simulink model "s20260910_config2torque_sim_chatgpt"  (R2025a)
settings: Solver=daessc  StartTime=0.0  StopTime=20  FixedStep=0.01  MaxStep=0.05  RelTol=1e-3  AbsTol=1e-3  EnableMultiTasking=on
undefined symbols (not defined in the file or in its folder): X, Y, Z
libraries: sm_lib x9, nesl_utility x4, snake_single_module_library_torque x1, slpidlib x1, simulink x1, spsSawtoothGeneratorLib x1, cstblocks x1
settings Model: Creator=dperera  LastModifiedBy=dperera
settings SolverCC: AutoScaleAbsTol=off  AlgebraicLoopSolver=TrustRegion  MaxZcPerStep=1.0
settings DataIOCC: LimitDataPoints=on  MaxDataPoints=10000
settings OptimizationCC: ReuseModelBlockBuffer=off  LifeSpan=inf
settings DebuggingCC: UnconnectedInputMsg=warning  UnconnectedOutputMsg=warning  UnconnectedLineMsg=warning  AllowSymbolicDim=off  SubsystemReferenceDiagnosticForUnitTest=warning  SFUnexpectedBacktrackingDiag=warning  SFNoUnconditionalDefaultTransitionDiag=warning  SFExecutionAtInitializationDiag=none  ArithmeticOperatorsInVariantConditions=warning
settings ModelReferenceCC: EnableRefExpFcnMdlSchedulingChecks=on
settings SFSimCC: SimUseLocalCustomCode=off  CustomCodeUndefinedFunction=UseInterfaceOnly
settings RTWCC: RTWUseLocalCustomCode=off  GPUComputeCapability=3.5  DLArmComputeVersion=19.05
settings CodeAppCC: StateflowObjectComments=on
settings GRTTargetCC: TargetLangStandard=C89/C90 (ANSI)
settings ConfigComp: CovMetricSettings=dw  CovSaveCumulativeToWorkspaceVar=on  CovSaveSingleToWorkspaceVar=on  CovExternalEMLEnable=off  CovSFcnEnable=off
settings SimscapeCC: SimscapeLogType=all  SimscapeLogSimulationStatistics=on  SimscapeLogDataHistory=10000.0

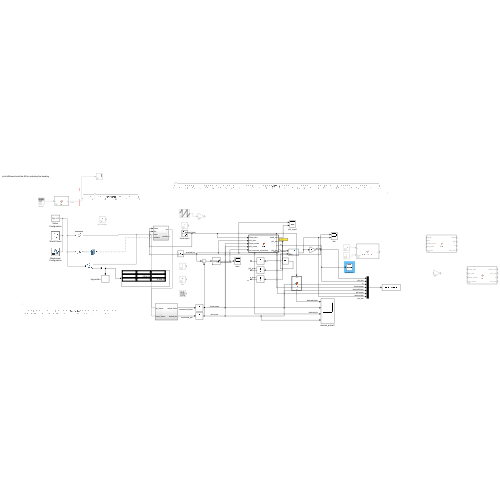
[thumbnail: Simulink's stored preview of the top-level diagram]
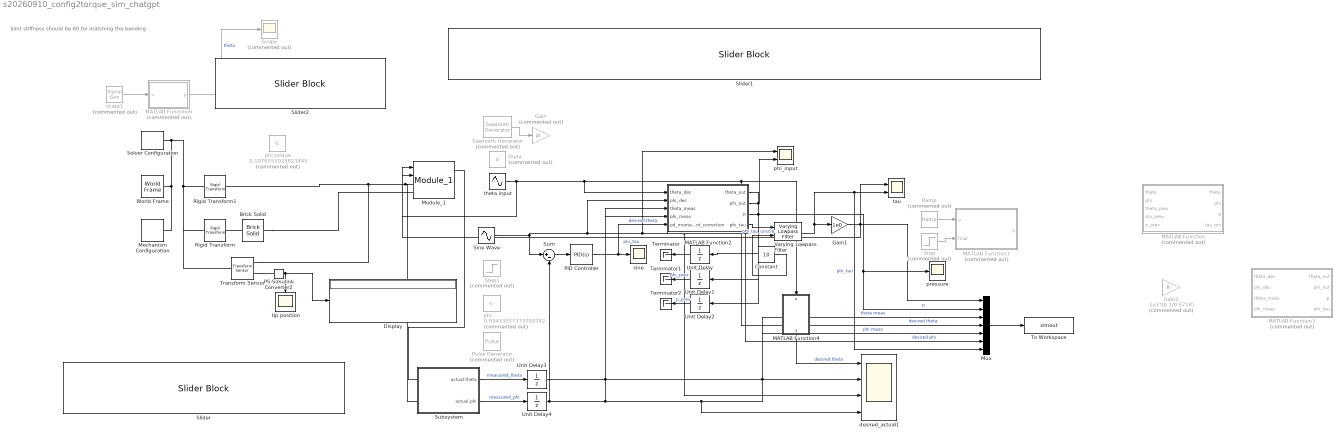
== system s20260910_config2torque_sim_chatgpt ==
  note: joint stiffness should be 60 for matching the bending
  Brick Solid : sm_lib/Body Elements/Brick Solid  BrickDimensions=[0.5 0.5 0.01]  BrickDimensionsUnits=m  ExportEntireGeometry=on  InertiaType=CalculateFromGeometry  BasedOnType=Density  Density=1000  DensityUnits=kg/m^3  Mass=1  MassUnits=kg  CenterOfMass=[0 0 0]  CenterOfMassUnits=m  MomentsOfInertia=[1 1 1]  MomentsOfInertiaUnits=kg*m^2  ProductsOfInertia=[0 0 0]  ProductsOfInertiaUnits=kg*m^2  GraphicType=FromGeometry  MarkerShape=Sphere  MarkerSize=10  GraphicVisPropType=SimpleVisualProperties  GraphicDiffuseColor=[0.5 0.5 0.5]  GraphicOpacity=1  GraphicSpecularColor=[0.5 0.5 0.5 1.0]  GraphicAmbientColor=[0.15 0.15 0.15 1.0]  GraphicEmissiveColor=[0.0 0.0 0.0 1.0]  GraphicShininess=75  DoExposeReferenceFrame=on  SerializedFrames=<Frames/>
  Constant : Constant  Value=10
  Display : Display
  Gain : Gain  Commented=on  Gain=pi
  Gain1 : Gain  Gain=1e0
  Gain2 : Gain  Commented=on  Gain=1e1*(0.1/0.5714)
  MATLAB Function : MATLAB Function  Commented=on  TreatAsAtomicUnit=on
  MATLAB Function1 : MATLAB Function  Commented=on  TreatAsAtomicUnit=on
  MATLAB Function2 : MATLAB Function  TreatAsAtomicUnit=on
  MATLAB Function3 : MATLAB Function  Commented=on  TreatAsAtomicUnit=on
  MATLAB Function4 : MATLAB Function  TreatAsAtomicUnit=on
  MATLAB Function6 : MATLAB Function  Commented=on  TreatAsAtomicUnit=on
  Mechanism Configuration : sm_lib/Utilities/Mechanism Configuration  UniformGravity=Constant  GravityVector=[0 0 -9.80665]  GravityVectorUnits=m/s^2  LinearizationDelta=0.001  JointModeTransitionNonlinearIterations=2
  Module_1 : snake_single_module_library_torque/Module_1  SystemSampleTime=-1  VariantActivationTime=update diagram  EmptyChoice=off  PassThrough=off  PassThroughVariantControl=(default)  EmptyChoiceVariantControl=(default)  AllowFlexibleInterface=on  Latency=0  AutoFrameSizeCalculation=off
  Mux : Mux  Inputs=7
  PID Controller : slpidlib/PID Controller  Controller=PID  Form=Parallel  TimeDomain=Continuous-time  UseExternalTs=off  SampleTime=-1  IntegratorMethod=Forward Euler  FilterMethod=Forward Euler  ControllerParametersSource=internal  P=0.3  I=0.1  UseKiTs=off  D=0.0001  UseExternalDerivativeSource=off  N=100  UseFilter=on  TunerSelectOption=Frequency Response Based  InitialConditionSource=internal  InitialConditionForIntegrator=0  InitialConditionForFilter=0  DifferentiatorICPrevScaledInput=0  ExternalReset=none  TrackingMode=off  Kt=1  LimitOutput=on  SatLimitsSource=internal  UpperSaturationLimit=inf  LowerSaturationLimit=-inf  LinearizeAsGain=on  AntiWindupMode=back-calculation  Kb=1  LimitIntegrator=off  UpperIntegratorSaturationLimit=inf  LowerIntegratorSaturationLimit=-inf  POutMin=[]  POutMax=[]  IOutMin=[]  IOutMax=[]  DOutMin=[]  DOutMax=[]  NOutMin=[]  NOutMax=[]  SumOutMin=[]  SumOutMax=[]  SaturationOutMin=[]  SaturationOutMax=[]  PParamMin=[]  PParamMax=[]  IParamMin=[]  IParamMax=[]  DParamMin=[]  DParamMax=[]  NParamMin=[]  NParamMax=[]  KbParamMin=[]  KbParamMax=[]  KtParamMin=[]  KtParamMax=[]  KbOutMin=[]  KbOutMax=[]  KtOutMin=[]  KtOutMax=[]  IntegratorOutMin=[]  IntegratorOutMax=[]  FilterOutMin=[]  FilterOutMax=[]  SumI1OutMin=[]  SumI1OutMax=[]  SumI2OutMin=[]  SumI2OutMax=[]  SumI3OutMin=[]  SumI3OutMax=[]  SumI4OutMin=[]  SumI4OutMax=[]  SumDOutMin=[]  SumDOutMax=[]  DifferentiatorOutMin=[]  DifferentiatorOutMax=[]  FilterDiffOutCoefMin=[]  FilterDiffOutCoefMax=[]  ReciprocalOutMin=[]  ReciprocalOutMax=[]  SumDenOutMin=[]  SumDenOutMax=[]  SumNumOutMin=[]  SumNumOutMax=[]  DivideOutMin=[]  DivideOutMax=[]  UdiffTsProdOutMin=[]  UdiffTsProdOutMax=[]  NTsProdOutMin=[]  NTsProdOutMax=[]  UintegralTsProdOutMin=[]  UintegralTsProdOutMax=[]  UngainTsProdOutMin=[]  UngainTsProdOutMax=[]  ClampingZeroOutDataTypeStr=Inherit: Inherit via back propagation  ClampingZeroOutMin=[]  ClampingZeroOutMax=[]  FilterDenConstantOutDataTypeStr=Inherit: Inherit via back propagation  FilterDenConstantOutMin=[]  FilterDenConstantOutMax=[]  PCopyOutDataTypeStr=Inherit: Inherit via back propagation  PCopyOutMin=[]  PCopyOutMax=[]  NCopyOutDataTypeStr=Inherit: Inherit via back propagation  NCopyOutMin=[]  NCopyOutMax=[]  IntegratorContinuousStateAttributes=''  IntegratorStateMustResolveToSignalObject=off  IntegratorRTWStateStorageClass=Auto  FilterContinuousStateAttributes=''  FilterStateMustResolveToSignalObject=off  FilterRTWStateStorageClass=Auto  ParallelPVariant=InternalParameters  IdealPVariant=Disabled  IVariant=InternalParameters  DVariant=InternalParameters  IntegratorVariant=Continuous  SatVariant=Enabled  AWVariant=BackCalculation  PCopyVariant=Disabled  TRVariant=Disabled  FdbkBlocksVariant=Forward  IdealPFdbkVariant=Disabled  SatFdbkVariant=Disabled  DerivativeFilterVariant=ContFilter  NVariant=InternalParameters  NCopyVariant=Disabled  FilterICVariant=InternalICsFilter  IntegratorICVariant=InternalICs  ExternalResetVariant=Disabled  TRSumVariant=Passthrough  SumFdbkVariant=Disabled  SumVariant=Sum_PID  TsampFilterVariant=InternalTs  TsampNgainVariant=Passthrough  TsampIntegralVariant=Disabled_SignalSpec  ExternalSaturationOutDataTypeStr=Inherit: Same as second input  DerivativeSourceVariant=ErrorSignal  PreIntVariant=InternalPreInt
  PS-Simulink Converter2 : nesl_utility/PS-Simulink Converter  PhysicalDomain=network_engine_domain  SubClassName=ps_output  LeftPortType=input  RightPortType=output  PseudoPeriodic=off  Frequencies=[]  VectorFormat=inherit  Unit=inherit  AffineConversion=off
  Pulse Generator : DiscretePulseGenerator  Commented=on  PulseType=Time based  Amplitude=pi/3  Period=4  PulseWidth=50  PhaseDelay=1
  Ramp : simulink/Sources/Ramp  Commented=on  slope=0.01*2*pi  start=1  InitialOutput=0.001
  Rigid Transform : sm_lib/Frames and Transforms/Rigid Transform  RotationMethod=None  FollAlignAxisA=+X  BaseAlignAxisA=+Y  FollAlignAxisB=+Y  BaseAlignAxisB=+Z  RotationStandardAxis=+Z  RotationAngle=0  RotationAngleUnits=deg  RotationArbitraryAxis=[0 0 1]  RotationSequenceAxes=FollowerAxes  RotationSequence=XYX  RotationSequenceAngles=[0 0 0]  RotationSequenceAnglesUnits=deg  RotationMatrix=[1 0 0;0 1 0;0 0 1]  Quaternion=[1 0 0 0]  TranslationMethod=StandardAxis  TranslationCartesianOffset=[0 0 0]  TranslationCartesianOffsetUnits=m  TranslationStandardAxis=+Z  TranslationStandardOffset=-0.03  TranslationStandardOffsetUnits=m  TranslationROffset=0  TranslationROffsetUnits=m  TranslationThetaOffset=0  TranslationThetaOffsetUnits=deg  TranslationZOffset=0  TranslationZOffsetUnits=m
  Rigid Transform1 : sm_lib/Frames and Transforms/Rigid Transform  RotationMethod=StandardAxis  FollAlignAxisA=+X  BaseAlignAxisA=+Y  FollAlignAxisB=+Y  BaseAlignAxisB=+Z  RotationStandardAxis=+X  RotationAngle=-pi/2  RotationAngleUnits=rad  RotationArbitraryAxis=[0 0 1]  RotationSequenceAxes=FollowerAxes  RotationSequence=XYX  RotationSequenceAngles=[0 0 0]  RotationSequenceAnglesUnits=deg  RotationMatrix=[1 0 0;0 1 0;0 0 1]  Quaternion=[1 0 0 0]  TranslationMethod=StandardAxis  TranslationCartesianOffset=[0 0 0]  TranslationCartesianOffsetUnits=m  TranslationStandardAxis=+Z  TranslationStandardOffset=0.5  TranslationStandardOffsetUnits=m  TranslationROffset=0  TranslationROffsetUnits=m  TranslationThetaOffset=0  TranslationThetaOffsetUnits=deg  TranslationZOffset=0  TranslationZOffsetUnits=m
  Sawtooth Generator : spsSawtoothGeneratorLib/Sawtooth Generator  Commented=on  Freq=0.5  Phase=180  Ts=0.001
  Scope : Scope  Commented=on
      settings: ActiveDisplayYMinimum=-3.3334127281449564  ActiveDisplayYMaximum=3.1584952199962761
  Sine Wave : Sin  Amplitude=pi/2-0.3  Bias=pi/2-0.3  Phase=3*pi/2  SampleTime=0
  Slider : SliderBlock  ScaleMin=-3.14  ScaleMax=6
  Slider1 : SliderBlock  ScaleMax=3.14
  Slider2 : SliderBlock  ScaleMax=0.5
  Solver Configuration : nesl_utility/Solver Configuration  PhysicalDomain=network_engine_domain  SubClassName=solver  LeftPortType=input  RightPortType=generic  Tones=[]  Harmonics=[]  SimulateNoise=off  Profile=off  UseLocalSampling=off  EnableSwitchedLinearOptims=on  FrequencyDomain=off  UseCCode=off  RelTol=0.001  AbsTol=1e-06  MinStep=1e-09  ToWorkspace=off  RevertToSquareIcSolve=off  NumHomotopyIterations=100  PhasorMode=off  PhasorModeNumHarmonics=1  ConsistencySolver=NEWTON_XTOL_AFTER_FTOL  IndexReductionMethod=DerivativeReplacement  DoDC=off  ResidualTolerance=1e-09  ConsistencyTolSource=GLOBAL  ConsistencyAbsTol=0.001  ConsistencyRelTol=0.001  ConsistencyTolFactor=0.001  UseLocalSolver=off  LocalSolverChoice=NE_BACKWARD_EULER_ADVANCER  ResolveIndetEquations=on  FunctionEvalNumThread=1  LocalSolverSampleTime=0.001  DoFixedCost=off  MaxNonlinIter=3  MaxModeIter=2  ComputeImpulses=off  ImpulseIterations=2  LinearAlgebra=Sparse  LinearAlgebraNumThread=0  EquationFormulation=NE_TIME_EF  DelaysMemoryBudget=1024  AutomaticFiltering=on  FilteringTimeConstant=0.001  PartitionStorageMethod=AS_NEEDED  PartitionMemoryBudget=1024  PartitionMethod=FAST  MultibodyUseLocalSolver=off  MultibodyLocalSolverChoice=ODE1  MultibodyLocalSolverSampleTime=0.001
  Step : Step  Commented=on  Time=2  SampleTime=0
  Step1 : Step  Commented=on  After=pi/3  SampleTime=0
  Subsystem : Subsystem
  Sum : Sum  Inputs=|+-
  Terminator : Terminator
  Terminator1 : Terminator
  Terminator2 : Terminator
  To Workspace : ToWorkspace  VariableName=simout  SaveFormat=Timeseries  SampleTime=-1
      settings: Save2DSignal=2-D array (concatenate along first dimension)
  Transform Sensor : sm_lib/Frames and Transforms/Transform Sensor  MeasurementFrame=World  RotationSequence=XYX  SenseAngle=off  SenseAxis=off  SenseQ=off  SenseR=on  SenseRotationSequence=off  SenseOmegaX=off  SenseOmegaY=off  SenseOmegaZ=off  SenseOmega=off  SenseQDot=off  SenseRDot=off  SenseRotationSequenceDot=off  SenseAlphaX=off  SenseAlphaY=off  SenseAlphaZ=off  SenseAlpha=off  SenseQDDot=off  SenseRDDot=off  SenseX=off  SenseY=off  SenseZ=off  SenseXYZ=off  SenseRad=off  SenseAzim=off  SenseDist=off  SenseInc=off  SenseXDot=off  SenseYDot=off  SenseZDot=off  SenseXYZDot=off  SenseRadDot=off  SenseAzimDot=off  SenseDistDot=off  SenseIncDot=off  SenseXDDot=off  SenseYDDot=off  SenseZDDot=off  SenseXYZDDot=off  SenseRadDDot=off  SenseAzimDDot=off  SenseDistDDot=off  SenseIncDDot=off
  Unit Delay : UnitDelay  InitialCondition=[0]  SampleTime=-1  HasFrameUpgradeWarning=on
  Unit Delay1 : UnitDelay  InitialCondition=0.0001  SampleTime=-1  HasFrameUpgradeWarning=on
  Unit Delay2 : UnitDelay  InitialCondition=[0.0001;0.01;0.001]  SampleTime=-1  HasFrameUpgradeWarning=on
  Unit Delay3 : UnitDelay  InitialCondition=[0]  SampleTime=-1  HasFrameUpgradeWarning=on
  Unit Delay4 : UnitDelay  InitialCondition=0.0001  SampleTime=-1  HasFrameUpgradeWarning=on
  Varying Lowpass Filter : cstblocks/Linear Parameter Varying/Varying Lowpass Filter  N=1
  World Frame : sm_lib/Frames and Transforms/World Frame
  desired_actual1 : Scope  NumInputPorts=4
      settings: ActiveDisplayYMinimum=-0.37614430678155741  ActiveDisplayYMaximum=3.3852987610340177  DataLoggingVariableName=ScopeData7
  phi : Constant  Commented=on  Value=0.03433257333758742
  phi torque : Constant  Commented=on  Value=0.1076555023923445
  phi_input : Scope  NumInputPorts=2
      settings: ActiveDisplayYMinimum=-0.36834079509334744  ActiveDisplayYMaximum=3.3160671558401278  DataLoggingVariableName=ScopeData3
  pressure : Scope
      settings: ActiveDisplayYMinimum=-30741.22465781157  ActiveDisplayYMaximum=510004.6447710325  DataLoggingVariableName=ScopeData4
  sine : Scope
      settings: ActiveDisplayYMinimum=-0.41740703510045596  ActiveDisplayYMaximum=3.0703490190244911  DataLoggingVariableName=ScopeData2
  tau : Scope  NumInputPorts=2
      settings: ActiveDisplayYMinimum=-0.07521570426510249  ActiveDisplayYMaximum=0.65254070404289077
  theta : Constant  Commented=on  Value=0
  theta input : Sin  Amplitude=pi-0.1  Frequency=0.1  SampleTime=0
  theta1 : SignalGenerator  Commented=on  WaveForm=sawtooth  Amplitude=pi  Frequency=0.1*2*pi  Units=rad/sec  VectorParams1D=off
  tip position : Scope
      settings: ActiveDisplayYMinimum=-1.2500000000000002  ActiveDisplayYMaximum=1.2500000000000004  DataLoggingVariableName=ScopeData5
  wires:
  Sawtooth Generator/1 -> Gain/1
  theta1/1 -> MATLAB Function6/1(u)
  MATLAB Function6/1(y) -> Scope/1  "theta"
  MATLAB Function2/1(theta_out) -> Unit Delay/1
  MATLAB Function2/2(phi_out) -> Unit Delay1/1, phi_input/2
  MATLAB Function2/3(p) -> Mux/2, pressure/1, Unit Delay2/1  "p"
  theta input/1 -> Mux/4, MATLAB Function4/1(u), MATLAB Function2/1(theta_des), Module_1/1  "desired theta"
  Ramp/1 -> MATLAB Function1/1(u)
  Step/1 -> MATLAB Function1/2(final)
  MATLAB Function4/1(y) -> desired_actual1/1  "desired theta"
  Gain1/1 -> Module_1/2, Mux/1, tau/1  "phi_tau"
  Sine Wave/1 -> desired_actual1/3, Mux/6, phi_input/1, MATLAB Function2/2(phi_des), Sum/1  "desired phi"
  Subsystem/1(actual theta) -> Unit Delay3/1  "measured_theta"
  Subsystem/2(actual phi) -> Unit Delay4/1  "measured_phi"
  Mux/1 -> To Workspace/1
  PID Controller/1 -> MATLAB Function2/5(pd_moment_correction), sine/1  "desired theta"
  Unit Delay/1 -> Terminator/1
  Unit Delay1/1 -> Terminator1/1  "phi_prev"
  Unit Delay2/1 -> Terminator2/1  "p_prev"
  Unit Delay3/1 -> Mux/3, desired_actual1/2, MATLAB Function2/3(theta_meas)  "theta meas"
  Unit Delay4/1 -> Mux/5, desired_actual1/4, MATLAB Function2/4(phi_meas), Sum/2  "phi meas"
  Sum/1 -> PID Controller/1
  MATLAB Function2/4(phi_tau) -> Varying Lowpass Filter/1  "phi_tau_unscle"
  Varying Lowpass Filter/1 -> Mux/7, tau/2, Gain1/1  "phi_tau"
  Constant/1 -> Varying Lowpass Filter/2
  PS-Simulink Converter2/1 -> Display/1, tip position/1
  connections:
  World Frame/RConn1 -- Transform Sensor/LConn1 -- Rigid Transform/LConn1 -- Rigid Transform1/LConn1 -- Solver Configuration/RConn1 -- Mechanism Configuration/RConn1
  Brick Solid/RConn1 -- Rigid Transform/RConn1
  Module_1/LConn1 -- Transform Sensor/RConn1 -- Rigid Transform1/RConn1 -- Subsystem/LConn2
  Brick Solid/LConn1 -- Module_1/LConn2
  Subsystem/LConn1 -- Module_1/RConn1
  Transform Sensor/RConn2 -- PS-Simulink Converter2/LConn1

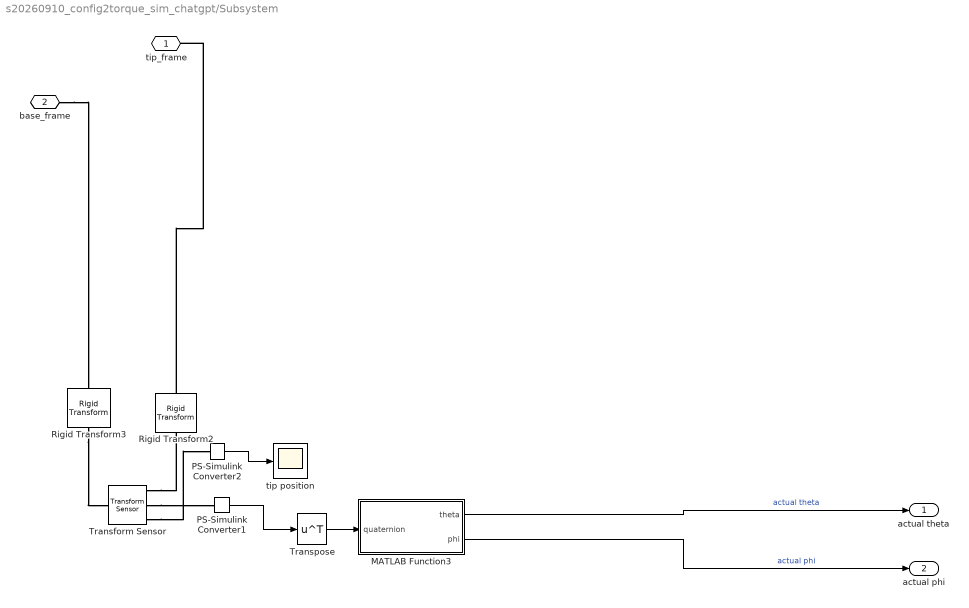
== system s20260910_config2torque_sim_chatgpt/Subsystem ==
  MATLAB Function3 : MATLAB Function  TreatAsAtomicUnit=on
  PS-Simulink Converter1 : nesl_utility/PS-Simulink Converter  PhysicalDomain=network_engine_domain  SubClassName=ps_output  LeftPortType=input  RightPortType=output  PseudoPeriodic=off  Frequencies=[]  VectorFormat=inherit  Unit=inherit  AffineConversion=off
  PS-Simulink Converter2 : nesl_utility/PS-Simulink Converter  PhysicalDomain=network_engine_domain  SubClassName=ps_output  LeftPortType=input  RightPortType=output  PseudoPeriodic=off  Frequencies=[]  VectorFormat=inherit  Unit=inherit  AffineConversion=off
  Rigid Transform2 : sm_lib/Frames and Transforms/Rigid Transform  RotationMethod=RotationSequence  FollAlignAxisA=+X  BaseAlignAxisA=+Y  FollAlignAxisB=+Y  BaseAlignAxisB=+Z  RotationStandardAxis=+Z  RotationAngle=pi  RotationAngleUnits=rad  RotationArbitraryAxis=[0 0 1]  RotationSequenceAxes=FollowerAxes  RotationSequence=XZY  RotationSequenceAngles=[-pi/2 pi 0]  RotationSequenceAnglesUnits=rad  RotationMatrix=[1 0 0;0 1 0;0 0 1]  Quaternion=[1 0 0 0]  TranslationMethod=None  TranslationCartesianOffset=[0 0 0]  TranslationCartesianOffsetUnits=m  TranslationStandardAxis=+Z  TranslationStandardOffset=-0.5  TranslationStandardOffsetUnits=m  TranslationROffset=0  TranslationROffsetUnits=m  TranslationThetaOffset=0  TranslationThetaOffsetUnits=deg  TranslationZOffset=0  TranslationZOffsetUnits=m
  Rigid Transform3 : sm_lib/Frames and Transforms/Rigid Transform  RotationMethod=RotationSequence  FollAlignAxisA=+X  BaseAlignAxisA=+Y  FollAlignAxisB=+Y  BaseAlignAxisB=+Z  RotationStandardAxis=+Z  RotationAngle=pi  RotationAngleUnits=rad  RotationArbitraryAxis=[0 0 1]  RotationSequenceAxes=FollowerAxes  RotationSequence=YXZ  RotationSequenceAngles=[pi -pi/2 0]  RotationSequenceAnglesUnits=rad  RotationMatrix=[1 0 0;0 1 0;0 0 1]  Quaternion=[1 0 0 0]  TranslationMethod=None  TranslationCartesianOffset=[0 0 0]  TranslationCartesianOffsetUnits=m  TranslationStandardAxis=+Z  TranslationStandardOffset=-0.5  TranslationStandardOffsetUnits=m  TranslationROffset=0  TranslationROffsetUnits=m  TranslationThetaOffset=0  TranslationThetaOffsetUnits=deg  TranslationZOffset=0  TranslationZOffsetUnits=m
  Transform Sensor : sm_lib/Frames and Transforms/Transform Sensor  MeasurementFrame=Follower  RotationSequence=XYZ  SenseAngle=off  SenseAxis=off  SenseQ=on  SenseR=off  SenseRotationSequence=off  SenseOmegaX=off  SenseOmegaY=off  SenseOmegaZ=off  SenseOmega=off  SenseQDot=off  SenseRDot=off  SenseRotationSequenceDot=off  SenseAlphaX=off  SenseAlphaY=off  SenseAlphaZ=off  SenseAlpha=off  SenseQDDot=off  SenseRDDot=off  SenseX=off  SenseY=off  SenseZ=off  SenseXYZ=on  SenseRad=off  SenseAzim=off  SenseDist=off  SenseInc=off  SenseXDot=off  SenseYDot=off  SenseZDot=off  SenseXYZDot=off  SenseRadDot=off  SenseAzimDot=off  SenseDistDot=off  SenseIncDot=off  SenseXDDot=off  SenseYDDot=off  SenseZDDot=off  SenseXYZDDot=off  SenseRadDDot=off  SenseAzimDDot=off  SenseDistDDot=off  SenseIncDDot=off
  Transpose : Math  Operator=transpose
  tip position : Scope
      settings: ActiveDisplayYMinimum=-0.036250000065594909  ActiveDisplayYMaximum=0.32625000000729432  DataLoggingVariableName=ScopeData6
  tip_frame : PMIOPort  Side=Left
  base_frame : PMIOPort  Port=2  Side=Left
  actual theta : Outport
  actual phi : Outport  Port=2
  wires:
  PS-Simulink Converter1/1 -> Transpose/1
  Transpose/1 -> MATLAB Function3/1(quaternion)
  MATLAB Function3/2(phi) -> actual phi/1  "actual phi"
  PS-Simulink Converter2/1 -> tip position/1
  MATLAB Function3/1(theta) -> actual theta/1  "actual theta"
  connections:
  Transform Sensor/RConn1 -- Rigid Transform2/RConn1
  Transform Sensor/RConn2 -- PS-Simulink Converter1/LConn1
  Rigid Transform3/RConn1 -- Transform Sensor/LConn1
  Transform Sensor/RConn3 -- PS-Simulink Converter2/LConn1
  base_frame/RConn1 -- Rigid Transform3/LConn1
  Rigid Transform2/LConn1 -- tip_frame/RConn1

== matlab function s20260910_config2torque_sim_chatgpt/MATLAB Function1 ==
  data: u input; y output; final input
function y = smoothStep(u, final)

y = u*(1-final);

if y <= 0.00001
    y= 0.001;
end

end

== matlab function s20260910_config2torque_sim_chatgpt/MATLAB Function ==
  data: theta input; theta output; phi input; theta_prev input; phi_prev input; p_prev input; phi output; p output; tau_phi output
function [theta, phi, p, tau_phi] = fcn(theta, phi, theta_prev, phi_prev, p_prev)
%#codegen 
% 
% This function computes torque required for the
% 
A = pi * (0.013/2)^2;
r = 0.013;
K = 0.00001;
N = 30;
L = 0.29;
l = L/N;

J_angle = f20260427_3_pressure2config_Jacobian(p_prev, A, K, r);
J_inv = pinv(J_angle);
% p = p_mat(:, i) + J_inv*([theta(i+1); phi(i+1)]-[frw(1,i); frw(2,i)]);
p = p_prev + J_inv*([theta; phi]-[theta_prev; phi_prev]);
% p = m20260427_5_PositivePressures(p);


[f, my, mx, ~, ~] = pressure2force_moment_config(p, A, r, K);
W = [mx; my; 0.0; 0.0; 0.0; f];
J = completeArm_Jacobian(theta_prev, phi_prev, l, N);

tau = J' * W;
tau_phi = tau(2);

== matlab function s20260910_config2torque_sim_chatgpt/MATLAB Function2 ==
  data: theta_des input; theta_out output; phi_des input; theta_meas input; phi_meas input; phi_out output; p output; phi_tau output; pd_moment_correction input
function [theta_out, phi_out, p, phi_tau] = ...
    fcn(theta_des, phi_des, theta_meas, phi_meas, pd_moment_correction)

%#codegen
%
% Inputs:
%   theta_des  : desired bending direction [rad]
%   phi_des    : desired total bending angle [rad]
%   theta_meas : measured bending direction [rad]
%   phi_meas   : measured total bending angle [rad]
%
% Outputs:
%   theta_out  : desired theta passed to the theta position controller
%   phi_out    : desired phi for logging
%   p          : calculated muscle pressures [Pa]
%   tau_phi    : first phi-joint torque [N*m]

%% Model parameters

A = pi*(0.013/2)^2;     % Muscle area [m^2]
r = 0.013;              % Muscle radial offset [m]
K = 0.19223750;            % Continuum bending stiffness [N*m/rad]

N = 29;                 % Number of rigid-link intervals
L = 0.29;               % Arm length [m]
l = L/N;                % Link length [m]

theta_out = theta_des;
phi_out = phi_des;


%% Desired bending moments

% my_des = K*phi_des*cos(theta_des);
% mx_des = -K*phi_des*sin(theta_des);

bending_moment_cmd = ...
    K*phi_des + pd_moment_correction;

my_des = bending_moment_cmd*cos(theta_des);
mx_des = -bending_moment_cmd*sin(theta_des);

%% Null-space pressure allocation

Ar = A*r;

% Differential pressures producing the desired moments.
% Their sum is zero.
p_delta = [ ...
    -2*my_des/(3*Ar);
     my_des/(3*Ar) + mx_des/(sqrt(3)*Ar);
     my_des/(3*Ar) - mx_des/(sqrt(3)*Ar)];

% Physical pressure limits
p_min = 0;          % [Pa]
p_max = 350000;     % 3.5 bar [Pa]

% Range of common pressure that satisfies all pressure limits
p_common_min = p_min - min(p_delta);
p_common_max = p_max - max(p_delta);

if p_common_min <= p_common_max

    % Desired bending moment is feasible.
    % Midpoint gives equal margin from the upper and lower limits.
    p_common = 0.5*(p_common_min + p_common_max);

    p = p_delta + p_common;

    moment_scale = 1.0;
    pressure_feasible = true;

else

    % Requested moment cannot be generated within the pressure limits.
    % Scale the differential pressures while preserving theta.
    pressure_span = max(p_delta) - min(p_delta);

    if pressure_span > 1e-12
        moment_scale = (p_max - p_min)/pressure_span;
    else
        moment_scale = 1.0;
    end

    p_delta = moment_scale*p_delta;

    % Recalculate the feasible common-pressure interval
    p_common_min = p_min - min(p_delta);
    p_common_max = p_max - max(p_delta);

    p_common = 0.5*(p_common_min + p_common_max);

    p = p_delta + p_common;

    pressure_feasible = false;

end

%% Recalculate achievable moments from allocated pressures

moment_y = -(A*r*(-p(2) - p(3) + 2*p(1)))/2;
moment_x = A*r*sqrt(3)*(p(2) - p(3))/2;

%% Moment-only tip wrench

W = [moment_x;
     moment_y;
     0;
     0;
     0;
     0];

%% Joint torque calculation

if abs(phi_meas) < 1e-6
    theta_for_J = theta_des;
else
    theta_for_J = theta_meas;
end

J = completeArm_Jacobian( ...
    theta_for_J, phi_meas, l, N);

tau = J.'*W;

phi_tau = tau(2);

end

== matlab function s20260910_config2torque_sim_chatgpt/Subsystem/MATLAB Function3 ==
  data: quaternion input; theta output; phi output
function [theta, phi] = IMU2Config(quaternion)
%#codegen
T = quat2rotm(quaternion);

theta= wrapToPi(atan2(T(2,3),T(1,3)));
phi= (acos(T(3,3)));

end

== matlab function s20260910_config2torque_sim_chatgpt/MATLAB Function4 ==
  data: u input; y output
function y = fcn(u)
%$codegen
y = wrapToPi(u);

== matlab function s20260910_config2torque_sim_chatgpt/MATLAB Function3 ==
  data: theta_des input; theta_out output; phi_des input; theta_meas input; phi_meas input; phi_out output; p output; phi_tau output
function [theta_out, phi_out, p, phi_tau] = ...
    fcn(theta_des, phi_des, theta_meas, phi_meas)

%#codegen
%
% Inputs:
%   theta_des  : desired bending direction [rad]
%   phi_des    : desired total bending angle [rad]
%   theta_meas : measured bending direction [rad]
%   phi_meas   : measured total bending angle [rad]
%
% Outputs:
%   theta_out  : desired theta passed to the theta position controller
%   phi_out    : desired phi for logging
%   p          : calculated muscle pressures [Pa]
%   tau_phi    : first phi-joint torque [N*m]

%% Model parameters

A = pi*(0.013/2)^2;     % Muscle area [m^2]
r = 0.013;              % Muscle radial offset [m]
K = 0.19223750;            % Continuum bending stiffness [N*m/rad]

N = 29;                 % Number of rigid-link intervals
L = 0.29;               % Arm length [m]
l = L/N;                % Link length [m]

theta_out = theta_des;
phi_out = phi_des;

%% Select the common pressure

% Maximum expected bending angle
phi_max = pi;

% Minimum common pressure required to prevent negative pressures.
% The factor 1.10 adds a 10% margin.
p_common = 1.10*(2*K*phi_max)/(3*A*r);

%% Direct configuration-to-pressure mapping

% Desired bending moments
my_des = K*phi_des*cos(theta_des);
mx_des = -K*phi_des*sin(theta_des);

Ar = A*r;

p1 = p_common - 2*my_des/(3*Ar);

p2 = p_common ...
   + my_des/(3*Ar) ...
   + mx_des/(sqrt(3)*Ar);

p3 = p_common ...
   + my_des/(3*Ar) ...
   - mx_des/(sqrt(3)*Ar);

p = [p1; p2; p3];

% Numerical protection. Adding the same pressure to all three muscles
% does not change the desired bending moments.
% minimum_pressure = min(p);
% 
% if minimum_pressure < 0
%     p = p - minimum_pressure;
% end

%% Calculate the tip wrench

% Corrected axial force
force_z = A*sum(p);

% Recalculate moments from the resulting pressures
moment_y = -(A*r*(-p(2) - p(3) + 2*p(1)))/2;
moment_x = A*r*sqrt(3)*(p(2) - p(3))/2;

% Tip-frame wrench:
% [Mx; My; Mz; Fx; Fy; Fz]
W = [moment_x;
     moment_y;
     0;
     0;
     0;
     0];

%% Calculate joint torques at the measured configuration

% Theta from a tip-pose estimator may be undefined when phi is almost zero.
% In that small region, use the commanded theta.
if abs(phi_meas) < 1e-6
    theta_for_J = theta_des;
else
    theta_for_J = theta_meas;
end

J = completeArm_Jacobian( ...
    theta_for_J, phi_meas, l, N);

tau = J.'*W;

% First phi joint. This preserves your current common-torque experiment.
phi_tau = tau(2);

end

== matlab function s20260910_config2torque_sim_chatgpt/MATLAB Function6 ==
  data: u input; y output
function y = fcn(u)

y = wrapToPi(u - pi);
